simulink model "Plant"  (R2018b)
settings: configuration reference "plant_config" (kept outside this file)
values from neighbouring files (symbols this model uses):
  ada =     [acdata.mat]    (also in aero_data.mat)
  ade =     [acdata.mat]    (also in aero_data.mat)
  adr =     [acdata.mat]    (also in aero_data.mat)
  adyn =     [acdata.mat]    (also in aero_data.mat)
  alat =     [acdata.mat]    (also in aero_data.mat)
  alon =     [acdata.mat]    (also in aero_data.mat)
  geo =     [acdata.mat]    (also in aero_data.mat)
  mc =     [acdata.mat]    (also in aero_data.mat)
  PLANT_EXPORT = Simulink.Parameter(PLANT_EXPORT_VALUE)    [plant_model_init.m]
  PLANT_PARAM = Simulink.Parameter(PLANT_PARAM_VALUE)    [plant_model_init.m]
undefined symbols (not defined in the file or in its folder): acc_x, acc_x_O, acc_y, acc_y_O, acc_z, acc_z_O, alt, alt_0, day, diff_pressure, DiscIntNeverNeededParam, fixType, flags, gSpeed, gyr_x, gyr_y, gyr_z, h_R, hAcc, heading, headingAcc, height, hMSL, hour, iTOW, lat, lon, M_BO, M_OB, mag_x, mag_y, mag_z, month, nano, numSV, pDOP, phi, PLANT_CONST, plant_model, pressure, prop_vel, psi, quat, reserved1, reserved2, rot_x_B, rot_y_B, rot_z_B, sAcc, sec, Sensor_Model, tAcc, temperature, temprature, theta, timestamp, Va, vAcc, valid, vel_x_O ... (+8)
libraries: FMT_Model_Lib x23, simulink x14, dspsrcs4 x6, aerolibatmos2 x1
(part 1 of 3)
settings Model: Creator=jc  LastModifiedBy=zouji
settings ConfigSetRef: SourceLocation=Base Workspace

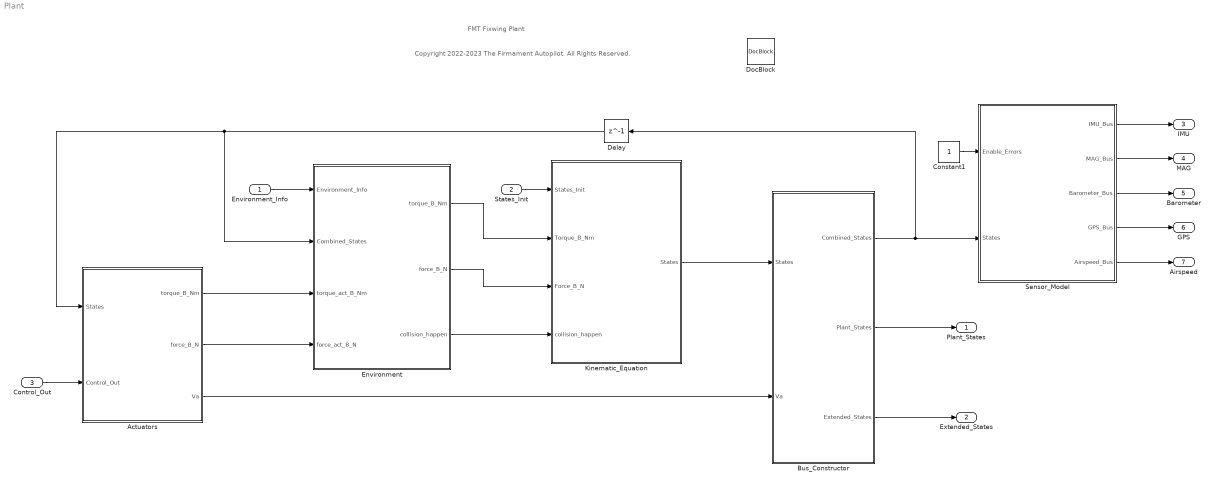
== system Plant ==
  note: FMT Fixwing Plant
  note: Copyright 2022-2023 The Firmament Autopilot. All Rights Reserved.
  Environment_Info : Inport  OutDataTypeStr=Bus: Environment_Info_Bus
  States_Init : Inport  Port=2  OutDataTypeStr=Bus: States_Init_Bus  Interpolate=off
  Control_Out : Inport  Port=3  OutDataTypeStr=Bus: Control_Out_Bus
  Actuators : Subsystem  TreatAsAtomicUnit=on
  Bus_Constructor : Subsystem  TreatAsAtomicUnit=on  mask{lat_0=PLANT_PARAM.LAT_0, lon_0=PLANT_PARAM.LON_0, hgt_0=PLANT_PARAM.ALT_0}
      mask prompts: lat_0 "init latitude (rad)"; lon_0 "init lontitude (rad)"; hgt_0 "init height (m)"
  Constant1 : Constant  OutDataTypeStr=Inherit: Inherit via back propagation
  Delay : Delay  DelayLength=1
  DocBlock : simulink/Model-Wide Utilities/DocBlock  DocumentType=Text
      content=|
      | This model is referenced from https://www.researchgate.net/publication/340630428_Guidance_and_control_for_a_fixed-wing_UAV
      | Aerodynamic data and models are contributed by pengyuan.shao@hotmail.com
  Environment : Subsystem  TreatAsAtomicUnit=on
  Kinematic_Equation : Subsystem  TreatAsAtomicUnit=on
  Sensor_Model : Subsystem  TreatAsAtomicUnit=on
  Plant_States : Outport  OutDataTypeStr=Bus: Plant_States_Bus
  Extended_States : Outport  Port=2  OutDataTypeStr=Bus: Extended_States_Bus
  IMU : Outport  Port=3  OutDataTypeStr=Bus: IMU_Bus
  MAG : Outport  Port=4  OutDataTypeStr=Bus: MAG_Bus
  Barometer : Outport  Port=5  OutDataTypeStr=Bus: Barometer_Bus
  GPS : Outport  Port=6  OutDataTypeStr=Bus: GPS_uBlox_Bus
  Airspeed : Outport  Port=7  OutDataTypeStr=Bus: AirSpeed_Bus
  wires:
  Environment/1(torque_B_Nm) -> Kinematic_Equation/2(Torque_B_Nm)
  Kinematic_Equation/1(States) -> Bus_Constructor/1(States)
  Actuators/2(force_B_N) -> Environment/4(force_act_B_N)
  Control_Out/1 -> Actuators/2(Control_Out)
  Actuators/1(torque_B_Nm) -> Environment/3(torque_act_B_Nm)
  Delay/1 -> Environment/2(Combined_States), Actuators/1(States)
  Environment/3(collision_happen) -> Kinematic_Equation/4(collision_happen)
  Environment/2(force_B_N) -> Kinematic_Equation/3(Force_B_N)
  Bus_Constructor/2(Plant_States) -> Plant_States/1
  Bus_Constructor/3(Extended_States) -> Extended_States/1
  Bus_Constructor/1(Combined_States) -> Delay/1, Sensor_Model/2(States)
  Sensor_Model/4(GPS_Bus) -> GPS/1
  Constant1/1 -> Sensor_Model/1(Enable_Errors)
  Sensor_Model/3(Barometer_Bus) -> Barometer/1
  Sensor_Model/2(MAG_Bus) -> MAG/1
  Sensor_Model/1(IMU_Bus) -> IMU/1
  Actuators/3(Va) -> Bus_Constructor/2(Va)
  Sensor_Model/5(Airspeed_Bus) -> Airspeed/1
  Environment_Info/1 -> Environment/1(Environment_Info)
  States_Init/1 -> Kinematic_Equation/1(States_Init)

== system Plant/Actuators ==
  States : Inport
  Control_Out : Inport  Port=2
  Aerodynamics Forces and Moments : Subsystem
  Propulsion Forces and Moments : Subsystem
  Reshape : Reshape  OutputDimensionality=Column vector (2-D)
  Reshape1 : Reshape  OutputDimensionality=Column vector (2-D)
  Sum : Sum  Inputs=|++
  Sum1 : Sum  Inputs=|++
  Wind_Triangle : Subsystem
  selector : Subsystem
  torque_B_Nm : Outport
  force_B_N : Outport  Port=2
  Va : Outport  Port=3
  wires:
  Control_Out/1 -> Aerodynamics Forces and Moments/5(Control_Out), Propulsion Forces and Moments/1(Control_Out)
  States/1 -> selector/1(States), Wind_Triangle/1(States)
  Wind_Triangle/1(Va) -> Aerodynamics Forces and Moments/1(Va_B), Va/1
  Wind_Triangle/2(alpha) -> Aerodynamics Forces and Moments/2(alpha)
  Wind_Triangle/3(beta) -> Aerodynamics Forces and Moments/3(beta)
  Aerodynamics Forces and Moments/2(Moment_B) -> Sum/1
  Propulsion Forces and Moments/2(Moment_B) -> Sum/2
  Sum/1 -> Reshape1/1
  Sum1/1 -> Reshape/1
  Aerodynamics Forces and Moments/1(Force_B) -> Sum1/1
  Propulsion Forces and Moments/1(Force_B) -> Sum1/2  "motor_force"
  Reshape/1 -> force_B_N/1
  Reshape1/1 -> torque_B_Nm/1
  selector/1(pqr) -> Aerodynamics Forces and Moments/4(pqr)

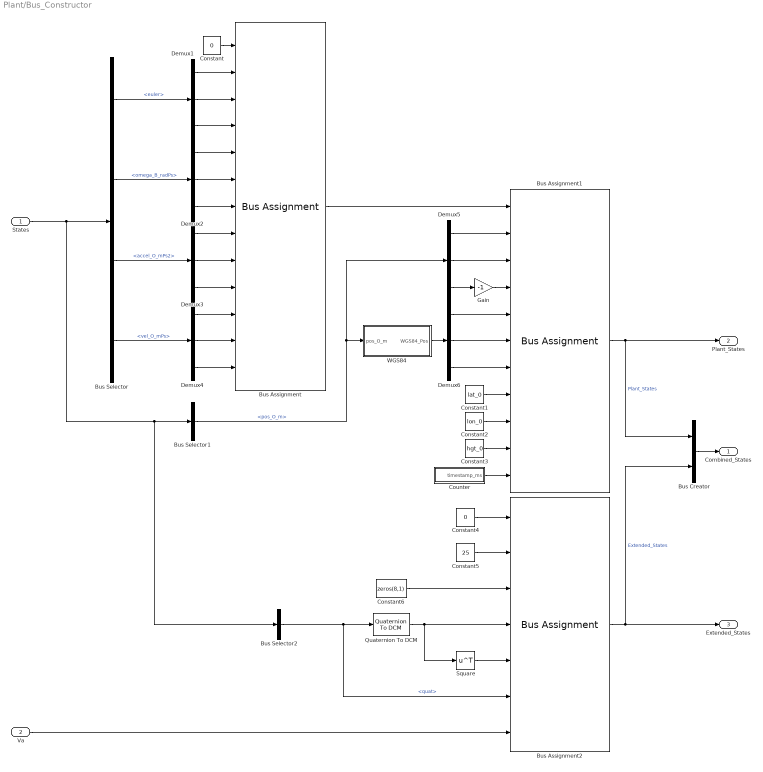
== system Plant/Bus_Constructor ==
  States : Inport
  Va : Inport  Port=2
  Bus Assignment : BusAssignment  AssignedSignals=phi,theta,psi,rot_x_B,rot_y_B,rot_z_B,acc_x_O,acc_y_O,acc_z_O,vel_x_O,vel_y_O,vel_z_O
  Bus Assignment1 : BusAssignment  AssignedSignals=x_R,y_R,h_R,lat,lon,alt,lat_0,lon_0,alt_0,timestamp
  Bus Assignment2 : BusAssignment  AssignedSignals=temprature,prop_vel,M_BO,M_OB,quat,Va
  Bus Creator : BusCreator  Inputs=2
  Bus Selector : BusSelector  OutputSignals=euler,omega_B_radPs,accel_O_mPs2,vel_O_mPs
  Bus Selector1 : BusSelector  OutputSignals=pos_O_m
  Bus Selector2 : BusSelector  OutputSignals=quat
  Constant : Constant  Value=0  OutDataTypeStr=Bus: Plant_States_Bus
  Constant1 : Constant  Value=lat_0
  Constant2 : Constant  Value=lon_0
  Constant3 : Constant  Value=hgt_0
  Constant4 : Constant  Value=0  OutDataTypeStr=Bus: Extended_States_Bus
  Constant5 : Constant  Value=25  OutDataTypeStr=Inherit: Inherit via back propagation
  Constant6 : Constant  Value=zeros(8,1)  OutDataTypeStr=single
  Counter : Subsystem
  Demux{1..6} (6 alike) : Demux  Outputs=3
  Gain : Gain  Gain=-1  OutDataTypeStr=Inherit: Same as input
  Quaternion To DCM : FMT_Model_Lib/Quaternion/Quaternion To DCM
      settings: SourceProductName=FMT Toolbox
  Square : Math  Operator=transpose  SaturateOnIntegerOverflow=on
  WGS84 : Subsystem
  Combined_States : Outport
  Plant_States : Outport  Port=2
  Extended_States : Outport  Port=3
  wires:
  Constant/1 -> Bus Assignment/1
  States/1 -> Bus Selector2/1, Bus Selector1/1, Bus Selector/1
  Bus Selector/1 -> Demux1/1  "<euler>"
  Bus Selector/2 -> Demux2/1  "<omega_B_radPs>"
  Bus Selector/3 -> Demux3/1  "<accel_O_mPs2>"
  Bus Selector/4 -> Demux4/1  "<vel_O_mPs>"
  Bus Assignment/1 -> Bus Assignment1/1
  Bus Selector1/1 -> Demux5/1, WGS84/1(pos_O_m)  "<pos_O_m>"
  Bus Assignment1/1 -> Plant_States/1, Bus Creator/1  "Plant_States"
  Demux1/2 -> Bus Assignment/3
  Demux5/3 -> Gain/1
  WGS84/1(WGS84_Pos) -> Demux6/1
  Demux1/1 -> Bus Assignment/2
  Demux1/3 -> Bus Assignment/4
  Demux2/1 -> Bus Assignment/5
  Demux2/2 -> Bus Assignment/6
  Demux2/3 -> Bus Assignment/7
  Demux3/1 -> Bus Assignment/8
  Demux3/2 -> Bus Assignment/9
  Demux3/3 -> Bus Assignment/10
  Demux4/1 -> Bus Assignment/11
  Demux4/2 -> Bus Assignment/12
  Demux4/3 -> Bus Assignment/13
  Demux5/2 -> Bus Assignment1/3
  Gain/1 -> Bus Assignment1/4
  Demux5/1 -> Bus Assignment1/2
  Demux6/1 -> Bus Assignment1/5
  Demux6/2 -> Bus Assignment1/6
  Demux6/3 -> Bus Assignment1/7
  Constant2/1 -> Bus Assignment1/9
  Constant1/1 -> Bus Assignment1/8
  Constant3/1 -> Bus Assignment1/10
  Constant4/1 -> Bus Assignment2/1
  Constant5/1 -> Bus Assignment2/2
  Constant6/1 -> Bus Assignment2/3
  Bus Selector2/1 -> Quaternion To DCM/1, Bus Assignment2/6  "<quat>"
  Bus Assignment2/1 -> Bus Creator/2, Extended_States/1  "Extended_States"
  Bus Creator/1 -> Combined_States/1
  Counter/1(timestamp_ms) -> Bus Assignment1/11
  Square/1 -> Bus Assignment2/5
  Quaternion To DCM/1 -> Square/1, Bus Assignment2/4
  Va/1 -> Bus Assignment2/7

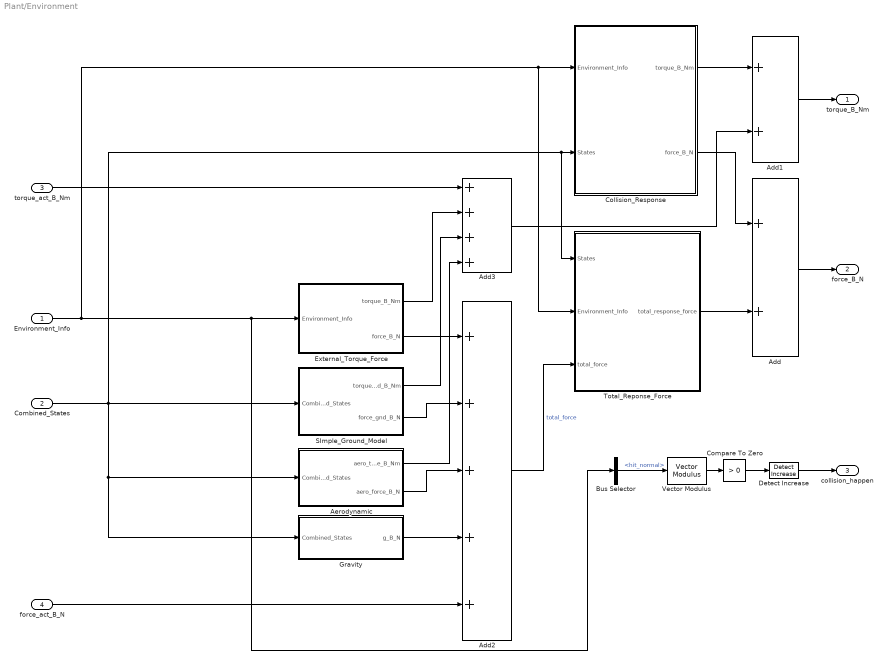
== system Plant/Environment ==
  Environment_Info : Inport
  Combined_States : Inport  Port=2
  torque_act_B_Nm : Inport  Port=3
  force_act_B_N : Inport  Port=4
  Add : Sum
  Add1 : Sum
  Add2 : Sum  Inputs=+++++
  Add3 : Sum  Inputs=++++
  Aerodynamic : Subsystem
  Bus Selector : BusSelector  OutputSignals=hit_normal
  Collision_Response : Subsystem  mask{e=0.5, u=1, Ixx=plant_model.Jxx, Iyy=plant_model.Jyy, Izz=plant_model.Jzz, m=plant_model.mass, dt=PLANT_CONST.dt}
      mask prompts: e "restitution coefficient [0 1]"; u "friction coefficient [0 1]"; m "mass (kg)"; dt "period (s)"
  Compare To Zero : simulink/Logic and Bit Operations/Compare To Zero  relop=>  OutDataTypeStr=boolean
  Detect Increase : simulink/Logic and Bit Operations/Detect Increase  vinit=0.0  OutDataTypeStr=boolean
  External_Torque_Force : Subsystem
  Gravity : Subsystem
  SImple_Ground_Model : Subsystem
  Total_Reponse_Force : Subsystem
  Vector Modulus : FMT_Model_Lib/Math/Vector Modulus
      settings: SourceProductName=FMT Toolbox
  torque_B_Nm : Outport
  force_B_N : Outport  Port=2
  collision_happen : Outport  Port=3
  wires:
  Add/1 -> force_B_N/1
  torque_act_B_Nm/1 -> Add3/1
  Add1/1 -> torque_B_Nm/1
  Combined_States/1 -> SImple_Ground_Model/1(Combined_States), Total_Reponse_Force/1(States), Collision_Response/2(States), Gravity/1(Combined_States), Aerodynamic/1(Combined_States)
  External_Torque_Force/2(force_B_N) -> Add2/1
  SImple_Ground_Model/2(force_gnd_B_N) -> Add2/2
  Gravity/1(g_B_N) -> Add2/4
  Aerodynamic/2(aero_force_B_N) -> Add2/3
  force_act_B_N/1 -> Add2/5
  SImple_Ground_Model/1(torque_gnd_B_Nm) -> Add3/3
  External_Torque_Force/1(torque_B_Nm) -> Add3/2
  Total_Reponse_Force/1(total_response_force) -> Add/2
  Add2/1 -> Total_Reponse_Force/3(total_force)  "total_force"
  Collision_Response/2(force_B_N) -> Add/1
  Add3/1 -> Add1/2
  Collision_Response/1(torque_B_Nm) -> Add1/1
  Aerodynamic/1(aero_torque_B_Nm) -> Add3/4
  Compare To Zero/1 -> Detect Increase/1
  Environment_Info/1 -> Bus Selector/1, External_Torque_Force/1(Environment_Info), Total_Reponse_Force/2(Environment_Info), Collision_Response/1(Environment_Info)
  Vector Modulus/1 -> Compare To Zero/1
  Bus Selector/1 -> Vector Modulus/1  "<hit_normal>"
  Detect Increase/1 -> collision_happen/1

== system Plant/Kinematic_Equation ==
  States_Init : Inport
  Torque_B_Nm : Inport  Port=2
  Force_B_N : Inport  Port=3
  collision_happen : Inport  Port=4
  Attitude_Dynamic : Subsystem  mask{Ixx=plant_model.Jxx, Iyy=plant_model.Jyy, Izz=plant_model.Jzz}
  Bus Creator : BusCreator  Inputs=7
  Constant : Constant  Value=0  OutDataTypeStr=Inherit: Inherit via back propagation
  Position_Dynamic : Subsystem  mask{mass=plant_model.mass}
  States : Outport
  wires:
  Attitude_Dynamic/2(omega_B_radPs) -> Position_Dynamic/2(omega_B_radPs), Bus Creator/2  "omega_B_radPs"
  Attitude_Dynamic/3(quat) -> Position_Dynamic/3(quat), Bus Creator/3  "quat"
  collision_happen/1 -> Position_Dynamic/4(vel_reset)
  Bus Creator/1 -> States/1  "states"
  Attitude_Dynamic/1(dot_omega_B_radPs2) -> Bus Creator/1  "dot_omega_B_radPs2"
  Attitude_Dynamic/4(euler) -> Bus Creator/4  "euler"
  Position_Dynamic/1(accel_O_mPs2) -> Bus Creator/5  "accel_O_mPs2"
  Position_Dynamic/2(vel_O_mPs) -> Bus Creator/6  "vel_O_mPs"
  Position_Dynamic/3(pos_O_m) -> Bus Creator/7  "pos_O_m"
  Force_B_N/1 -> Position_Dynamic/1(force_B_N)
  Torque_B_Nm/1 -> Attitude_Dynamic/1(torque_B_Nm)
  Constant/1 -> Attitude_Dynamic/2(rate_reset)
  States_Init/1 -> Position_Dynamic/5(States_Init), Attitude_Dynamic/3(States_Init)

== system Plant/Sensor_Model ==
  Enable_Errors : Inport  OutDataTypeStr=uint8
  States : Inport  Port=2
  Counter : Subsystem
  Sensor_Airspeed : Subsystem  TreatAsAtomicUnit=on
  Sensor_Barometer : Subsystem  TreatAsAtomicUnit=on
  Sensor_GPS : Subsystem  TreatAsAtomicUnit=on
  Sensor_IMU : Subsystem  TreatAsAtomicUnit=on
  Sensor_MAG : Subsystem  TreatAsAtomicUnit=on
  IMU_Bus : Outport
  MAG_Bus : Outport  Port=2
  Barometer_Bus : Outport  Port=3
  GPS_Bus : Outport  Port=4
  Airspeed_Bus : Outport  Port=5
  wires:
  Counter/1(timestamp_ms) -> Sensor_Airspeed/3(timestamp_ms), Sensor_Barometer/3(timestamp_ms), Sensor_MAG/3(timestamp_ms), Sensor_IMU/3(timestamp_ms), Sensor_GPS/3(timestamp_ms)
  States/1 -> Sensor_Airspeed/1(States), Sensor_GPS/1(States), Sensor_Barometer/1(States), Sensor_MAG/1(States), Sensor_IMU/1(States)
  Sensor_Barometer/1(Barometer_Bus) -> Barometer_Bus/1
  Sensor_MAG/1(MAG_Bus) -> MAG_Bus/1
  Sensor_IMU/1(IMU_Bus) -> IMU_Bus/1
  Enable_Errors/1 -> Sensor_IMU/2(Enable_Errors), Sensor_Airspeed/2(Enable_Errors), Sensor_GPS/2(Enable_Errors), Sensor_Barometer/2(Enable_Errors), Sensor_MAG/2(Enable_Errors)
  Sensor_GPS/1(GPS_Bus) -> GPS_Bus/1
  Sensor_Airspeed/1(Airspeed_Bus) -> Airspeed_Bus/1

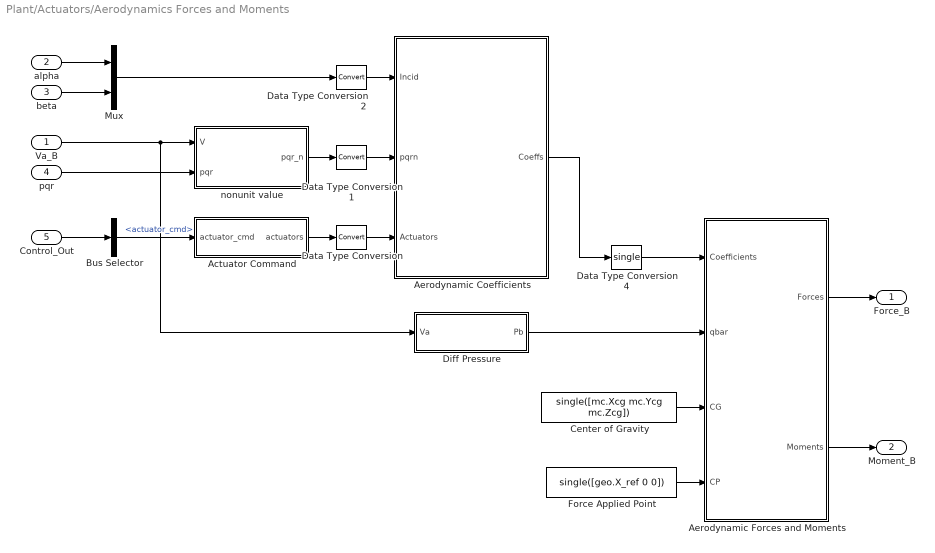
== system Plant/Actuators/Aerodynamics Forces and Moments ==
  Va_B : Inport
  alpha : Inport  Port=2
  beta : Inport  Port=3
  pqr : Inport  Port=4
  Control_Out : Inport  Port=5
  Actuator Command : Subsystem
  Aerodynamic Coefficients : Subsystem
  Aerodynamic Forces and Moments : Subsystem  mask(Aerodynamic Forces and Moments){S=geo.Sw, b=geo.b, cbar=geo.MAC}
      mask prompts: S "Reference area:"; b "Reference span:"; cbar "Reference length:"
      mask help: Compute the aerodynamic forces and moments applied at the center of gravity using the aerodynamic coefficients, dynamic pressure, center of gravity and center of pressure.
      mask Help: web(asbhelp);
      mask Display:
      | port_label('input',1,'Coefficients','texmode','on');
      | port_label('input',2,'q_{bar}','texmode','on');
      | port_label('input',3,'CG','texmode','on');
      | port_label('input',4,'CP','texmode','on');
      | port_label('output',1,'F_{aero}','texmode','on');
      | port_label('output',2,'M_{aero}','texmode','on');
  Bus Selector : BusSelector  OutputSignals=actuator_cmd
  Center of Gravity : Constant  Value=single([mc.Xcg mc.Ycg mc.Zcg])
  Data Type Conversion : DataTypeConversion
  Data Type Conversion1 : DataTypeConversion
  Data Type Conversion2 : DataTypeConversion
  Data Type Conversion4 : DataTypeConversion  OutDataTypeStr=single
  Diff Pressure : Subsystem
  Force Applied Point : Constant  Value=single([geo.X_ref 0 0])
  Mux : Mux  Inputs=2
  nonunit value : Subsystem
  Force_B : Outport
  Moment_B : Outport  Port=2
  wires:
  Control_Out/1 -> Bus Selector/1
  nonunit value/1(pqr_n) -> Data Type Conversion1/1
  Mux/1 -> Data Type Conversion2/1
  alpha/1 -> Mux/1
  beta/1 -> Mux/2
  Va_B/1 -> Diff Pressure/1(Va), nonunit value/1(V)
  pqr/1 -> nonunit value/2(pqr)
  Bus Selector/1 -> Actuator Command/1(actuator_cmd)  "<actuator_cmd>"
  Actuator Command/1(actuators) -> Data Type Conversion/1
  Data Type Conversion/1 -> Aerodynamic Coefficients/3(Actuators)
  Data Type Conversion1/1 -> Aerodynamic Coefficients/2(pqrn)
  Data Type Conversion2/1 -> Aerodynamic Coefficients/1(Incid)
  Aerodynamic Coefficients/1(Coeffs) -> Data Type Conversion4/1
  Data Type Conversion4/1 -> Aerodynamic Forces and Moments/1(Coefficients)
  Aerodynamic Forces and Moments/2(Moments) -> Moment_B/1
  Aerodynamic Forces and Moments/1(Forces) -> Force_B/1
  Center of Gravity/1 -> Aerodynamic Forces and Moments/3(CG)
  Force Applied Point/1 -> Aerodynamic Forces and Moments/4(CP)
  Diff Pressure/1(Pb) -> Aerodynamic Forces and Moments/2(qbar)

== system Plant/Actuators/Propulsion Forces and Moments ==
  Control_Out : Inport
  Constant : Constant  Value=[0 0 0]  OutDataTypeStr=single
  ESCs : Subsystem  mask{T=plant_model.motorT, k=plant_model.motorCr, p=plant_model.motorWb}
  Force : Subsystem
  Force_B : Outport
  Moment_B : Outport  Port=2
  wires:
  ESCs/1(rotor_speed_radPs) -> Force/1(rotor_speed_radPs)
  Control_Out/1 -> ESCs/1(Control_Out)
  Constant/1 -> Moment_B/1
  Force/1(force_B_N) -> Force_B/1

== system Plant/Actuators/Wind_Triangle ==
  States : Inport
  Attack_Angle : Subsystem
  Bus Selector : BusSelector  OutputSignals=Plant_States.vel_x_O,Plant_States.vel_y_O,Plant_States.vel_z_O
  Bus Selector1 : BusSelector  OutputSignals=Extended_States.M_BO
  Multiply : Product  Multiplication=Matrix(*)
  Mux : Mux  Inputs=3
  Selector : Selector  InputPortWidth=3  IndexOptions=Index vector (dialog)  Indices=1  OutputSizes=1
  Slide_Angle : Subsystem
  Sum : Sum  Inputs=|+-
  Wind_Velocity_O : Constant  Value=[0;0;0]  VectorParams1D=off  OutDataTypeStr=single
  Va : Outport
  alpha : Outport  Port=2
  beta : Outport  Port=3
  wires:
  States/1 -> Bus Selector1/1, Bus Selector/1
  Bus Selector/1 -> Mux/1  "<vel_x_O>"
  Bus Selector/2 -> Mux/2  "<vel_y_O>"
  Bus Selector/3 -> Mux/3  "<vel_z_O>"
  Bus Selector1/1 -> Multiply/1  "<M_BO>"
  Multiply/1 -> Selector/1, Slide_Angle/1(Va_B), Attack_Angle/1(Va_B)  "Va_B"
  Attack_Angle/1(alpha_rad) -> alpha/1  "alpha_rad"
  Slide_Angle/1(beta_rad) -> beta/1  "beta_rad"
  Selector/1 -> Va/1
  Mux/1 -> Sum/1
  Sum/1 -> Multiply/2
  Wind_Velocity_O/1 -> Sum/2

== system Plant/Actuators/selector ==
  States : Inport
  Bus Selector : BusSelector  OutputSignals=Plant_States.rot_x_B,Plant_States.rot_y_B,Plant_States.rot_z_B
  Mux : Mux  Inputs=3
  pqr : Outport
  wires:
  Bus Selector/1 -> Mux/1  "<rot_x_B>"
  Bus Selector/3 -> Mux/3  "<rot_z_B>"
  Bus Selector/2 -> Mux/2  "<rot_y_B>"
  Mux/1 -> pqr/1
  States/1 -> Bus Selector/1

== system Plant/Bus_Constructor/Counter ==
  Data Type Conversion2 : DataTypeConversion  OutDataTypeStr=uint32
  Delay : Delay  DelayLength=1  InitialCondition=0
  Sum : Sum  Inputs=|++
  dt : Constant  Value=PLANT_EXPORT.period  OutDataTypeStr=uint32
  timestamp_ms : Outport
  wires:
  dt/1 -> Sum/1
  Sum/1 -> Delay/1
  Delay/1 -> Data Type Conversion2/1
  Data Type Conversion2/1 -> timestamp_ms/1, Sum/2

== system Plant/Bus_Constructor/WGS84 ==
  pos_O_m : Inport
  Add : Sum
  Constant1 : Constant  Value=lat_0
  Constant2 : Constant  Value=lon_0
  Constant3 : Constant  Value=hgt_0
  Data Type Conversion : DataTypeConversion  OutDataTypeStr=double
  Delay : Delay  DelayLength=1
  Delay1 : Delay  DelayLength=1  InitialConditionSource=Input port  InitialCondition=[lat_0;lon_0;hgt_0]
      settings: InputPortMap=u0,p4
  Demux : Demux  Outputs=3
  Divide : Product  Inputs=/*
  Mux : Mux  Inputs=3
  Mux1 : Mux  Inputs=3
  Subtract : Sum  Inputs=+-
  Terminator : Terminator
  WGS84_Derivative : Subsystem
  Zero_Value_Exclusion : Subsystem
  WGS84_Pos : Outport
  wires:
  pos_O_m/1 -> Data Type Conversion/1
  Delay/1 -> Subtract/2
  WGS84_Derivative/1(dx_dlat) -> Mux/1
  Mux/1 -> Zero_Value_Exclusion/1(u)
  Zero_Value_Exclusion/1(y) -> Divide/1
  WGS84_Derivative/3(dz_dh) -> Mux/3
  WGS84_Derivative/2(dy_dlon) -> Mux/2
  Subtract/1 -> Divide/2
  Divide/1 -> Add/1
  Delay1/1 -> Demux/1, Add/2
  Demux/1 -> WGS84_Derivative/1(lat_0)
  Demux/3 -> WGS84_Derivative/2(h_0)
  Demux/2 -> Terminator/1
  Data Type Conversion/1 -> Delay/1, Subtract/1
  Constant1/1 -> Mux1/1
  Mux1/1 -> Delay1/2
  Add/1 -> Delay1/1, WGS84_Pos/1
  Constant2/1 -> Mux1/2
  Constant3/1 -> Mux1/3

== system Plant/Environment/Aerodynamic ==
  Combined_States : Inport
  Air_Drag : Subsystem
  aero_torque_B_Nm : Outport
  aero_force_B_N : Outport  Port=2
  wires:
  Combined_States/1 -> Air_Drag/1(Combined_States)
  Air_Drag/2(airdrag_force_B) -> aero_force_B_N/1  "aero_force_B_N"
  Air_Drag/1(airdrag_torque_B) -> aero_torque_B_Nm/1  "aero_torque_B_N"

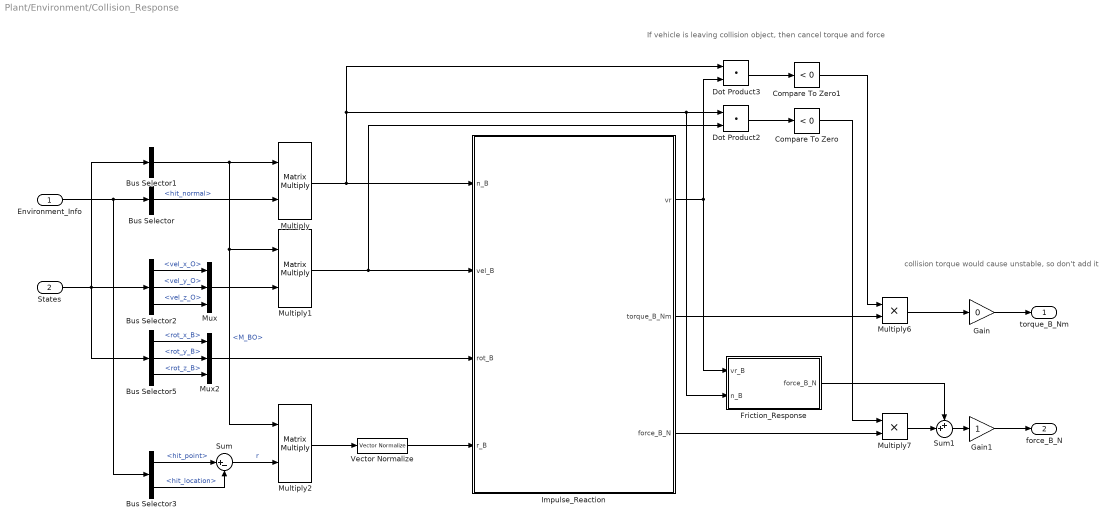
== system Plant/Environment/Collision_Response ==
  note: collision torque would cause unstable, so don't add it
  note: If vehicle is leaving collision object, then cancel torque and force
  Environment_Info : Inport
  States : Inport  Port=2
  Bus Selector : BusSelector  OutputSignals=hit_normal
  Bus Selector1 : BusSelector  OutputSignals=Extended_States.M_BO
  Bus Selector2 : BusSelector  OutputSignals=Plant_States.vel_x_O,Plant_States.vel_y_O,Plant_States.vel_z_O
  Bus Selector3 : BusSelector  OutputSignals=hit_point,hit_location
  Bus Selector5 : BusSelector  OutputSignals=Plant_States.rot_x_B,Plant_States.rot_y_B,Plant_States.rot_z_B
  Compare To Zero : simulink/Logic and Bit Operations/Compare To Zero  relop=<  OutDataTypeStr=boolean
  Compare To Zero1 : simulink/Logic and Bit Operations/Compare To Zero  relop=<  OutDataTypeStr=boolean
  Dot Product2 : DotProduct  InputSameDT=on  OutDataTypeStr=Inherit: Inherit via internal rule
  Dot Product3 : DotProduct  InputSameDT=on  OutDataTypeStr=Inherit: Inherit via internal rule
  Friction_Response : Subsystem
  Gain : Gain  Gain=0
  Gain1 : Gain
  Impulse_Reaction : Subsystem
  Multiply : Product  Multiplication=Matrix(*)
  Multiply1 : Product  Multiplication=Matrix(*)
  Multiply2 : Product  Multiplication=Matrix(*)
  Multiply6 : Product
  Multiply7 : Product
  Mux : Mux  Inputs=3
  Mux2 : Mux  Inputs=3
  Sum : Sum  Inputs=|+-
  Sum1 : Sum  Inputs=++|
  Vector Normalize : FMT_Model_Lib/Math/Vector Normalize
      settings: SourceProductName=FMT Toolbox
  torque_B_Nm : Outport
  force_B_N : Outport  Port=2
  wires:
  Environment_Info/1 -> Bus Selector3/1, Bus Selector/1
  Bus Selector/1 -> Multiply/2  "<hit_normal>"
  States/1 -> Bus Selector1/1, Bus Selector5/1, Bus Selector2/1
  Bus Selector1/1 -> Multiply/1, Multiply2/1, Multiply1/1  "<M_BO>"
  Bus Selector2/1 -> Mux/1  "<vel_x_O>"
  Bus Selector2/2 -> Mux/2  "<vel_y_O>"
  Bus Selector2/3 -> Mux/3  "<vel_z_O>"
  Mux/1 -> Multiply1/2
  Multiply1/1 -> Dot Product2/2, Impulse_Reaction/2(vel_B)
  Bus Selector3/1 -> Sum/1  "<hit_point>"
  Multiply2/1 -> Vector Normalize/1
  Bus Selector5/2 -> Mux2/2  "<rot_y_B>"
  Bus Selector5/3 -> Mux2/3  "<rot_z_B>"
  Bus Selector5/1 -> Mux2/1  "<rot_x_B>"
  Multiply/1 -> Dot Product2/1, Friction_Response/2(n_B), Dot Product3/1, Impulse_Reaction/1(n_B)
  Dot Product2/1 -> Compare To Zero/1
  Compare To Zero/1 -> Multiply7/1
  Multiply6/1 -> Gain/1
  Multiply7/1 -> Sum1/2
  Dot Product3/1 -> Compare To Zero1/1
  Compare To Zero1/1 -> Multiply6/1
  Bus Selector3/2 -> Sum/2  "<hit_location>"
  Sum/1 -> Multiply2/2  "r"
  Mux2/1 -> Impulse_Reaction/3(rot_B)
  Vector Normalize/1 -> Impulse_Reaction/4(r_B)
  Impulse_Reaction/1(vr) -> Dot Product3/2, Friction_Response/1(vr_B)
  Impulse_Reaction/2(torque_B_Nm) -> Multiply6/2
  Impulse_Reaction/3(force_B_N) -> Multiply7/2
  Friction_Response/1(force_B_N) -> Sum1/1
  Gain/1 -> torque_B_Nm/1
  Gain1/1 -> force_B_N/1
  Sum1/1 -> Gain1/1

== system Plant/Environment/External_Torque_Force ==
  Environment_Info : Inport
  Bus Selector : BusSelector  OutputSignals=torque,force
  torque_B_Nm : Outport
  force_B_N : Outport  Port=2
  wires:
  Environment_Info/1 -> Bus Selector/1
  Bus Selector/1 -> torque_B_Nm/1  "<torque>"
  Bus Selector/2 -> force_B_N/1  "<force>"

== system Plant/Environment/Gravity ==
  Combined_States : Inport
  Bus Selector4 : BusSelector  OutputSignals=Extended_States.M_BO
  Multiply3 : Product  Multiplication=Matrix(*)
  mg : Constant  Value=[0;0;9.81*plant_model.mass]  OutDataTypeStr=single
  g_B_N : Outport
  wires:
  Combined_States/1 -> Bus Selector4/1
  Bus Selector4/1 -> Multiply3/1  "<M_BO>"
  Multiply3/1 -> g_B_N/1
  mg/1 -> Multiply3/2

== system Plant/Environment/SImple_Ground_Model ==
  Combined_States : Inport
  Bus Selector : BusSelector  OutputSignals=Plant_States.h_R
  Compare To Zero : simulink/Logic and Bit Operations/Compare To Zero  relop=<  OutDataTypeStr=boolean
  Constant : Constant  Value=[0;0;0]  VectorParams1D=off  OutDataTypeStr=single
  Constant1 : Constant  Value=[0;0;0]  VectorParams1D=off  OutDataTypeStr=single
  Ground_Force : Subsystem
  Ground_Torque : Subsystem
  Switch1 : Switch  Criteria=u2 > Threshold
  Switch2 : Switch  Criteria=u2 > Threshold
  torque_gnd_B_Nm : Outport
  force_gnd_B_N : Outport  Port=2
  wires:
  Compare To Zero/1 -> Switch1/2, Switch2/2
  Constant/1 -> Switch2/3
  Switch2/1 -> force_gnd_B_N/1
  Combined_States/1 -> Ground_Force/1(Combined_States), Bus Selector/1, Ground_Torque/1(States)
  Bus Selector/1 -> Compare To Zero/1  "<h_R>"
  Ground_Force/1(force_gnd_B_N) -> Switch2/1
  Ground_Torque/1(torque_gnd_B_Nm) -> Switch1/1
  Constant1/1 -> Switch1/3
  Switch1/1 -> torque_gnd_B_Nm/1

== system Plant/Environment/Total_Reponse_Force ==
  States : Inport
  Environment_Info : Inport  Port=2
  total_force : Inport  Port=3
  Bus Selector : BusSelector  OutputSignals=hit_normal
  Bus Selector1 : BusSelector  OutputSignals=Extended_States.M_BO
  Compare To Zero : simulink/Logic and Bit Operations/Compare To Zero  relop=<  OutDataTypeStr=boolean
  Dot Product : DotProduct  InputSameDT=on  OutDataTypeStr=Inherit: Inherit via internal rule
  Multiply : Product  Multiplication=Matrix(*)
  Multiply1 : Product  Inputs=3
  Sum : Sum  Inputs=|+-
  total_response_force : Outport
  wires:
  total_force/1 -> Dot Product/1, Sum/1
  Bus Selector/1 -> Multiply/2  "<hit_normal>"
  Bus Selector1/1 -> Multiply/1  "<M_BO>"
  Multiply/1 -> Multiply1/3, Dot Product/2  "n_B"
  States/1 -> Bus Selector1/1
  Environment_Info/1 -> Bus Selector/1
  Multiply1/1 -> Sum/2
  Sum/1 -> total_response_force/1
  Compare To Zero/1 -> Multiply1/1
  Dot Product/1 -> Multiply1/2, Compare To Zero/1

== system Plant/Kinematic_Equation/Attitude_Dynamic ==
  torque_B_Nm : Inport
  rate_reset : Inport  Port=2
  States_Init : Inport  Port=3
  Bus Selector : BusSelector  OutputSignals=timestamp,euler
  Cross Product : FMT_Model_Lib/Math/Cross Product
      settings: SourceProductName=FMT Toolbox
  Detect Change : simulink/Logic and Bit Operations/Detect Change  vinit=0  OutDataTypeStr=boolean
  Discrete-Time Integrator : DiscreteIntegrator  ExternalReset=level  InitialCondition=[0;0;0]  SampleTime=-1  ICPrevOutput=DiscIntNeverNeededParam  ICPrevScaledInput=DiscIntNeverNeededParam
  Divide : Product  Inputs=/*  Multiplication=Matrix(*)  OutDataTypeStr=Inherit: Same as first input
  Euler To Quaternion : FMT_Model_Lib/Quaternion/Euler To Quaternion
      settings: SourceProductName=FMT Toolbox
  Inertia_Matrix : Constant  Value=[Ixx 0 0;0 Iyy 0;0 0 Izz]  OutDataTypeStr=single
  Logical Operator : Logic  Operator=OR  AllPortsSameDT=off  OutDataTypeStr=boolean
  Multiply : Product  Multiplication=Matrix(*)  OutDataTypeStr=Inherit: Same as first input
  Quaternion To Euler : FMT_Model_Lib/Quaternion/Quaternion To Euler
      settings: SourceProductName=FMT Toolbox
  Quaternuin_Update : Subsystem
  Sum : Sum  Inputs=|+-  OutDataTypeStr=Inherit: Same as first input
  dot_omega_B_radPs2 : Outport
  omega_B_radPs : Outport  Port=2
  quat : Outport  Port=3
  euler : Outport  Port=4
  wires:
  Quaternion To Euler/1 -> euler/1
  Quaternuin_Update/1(quat) -> Quaternion To Euler/1, quat/1
  rate_reset/1 -> Logical Operator/1
  Divide/1 -> dot_omega_B_radPs2/1, Discrete-Time Integrator/1  "dot_omega_B_radPs2"
  Sum/1 -> Divide/2
  Cross Product/1 -> Sum/2
  torque_B_Nm/1 -> Sum/1
  Multiply/1 -> Cross Product/2
  Inertia_Matrix/1 -> Multiply/1, Divide/1
  Discrete-Time Integrator/1 -> omega_B_radPs/1, Cross Product/1, Multiply/2, Quaternuin_Update/1(omega_B_radPs)  "omega_B_radPs"
  States_Init/1 -> Bus Selector/1
  Bus Selector/1 -> Detect Change/1  "<timestamp>"
  Logical Operator/1 -> Discrete-Time Integrator/2
  Detect Change/1 -> Quaternuin_Update/2(att_reset), Logical Operator/2
  Bus Selector/2 -> Euler To Quaternion/1  "<euler>"
  Euler To Quaternion/1 -> Quaternuin_Update/3(quat_0)

== system Plant/Kinematic_Equation/Position_Dynamic ==
  force_B_N : Inport
  omega_B_radPs : Inport  Port=2
  quat : Inport  Port=3
  vel_reset : Inport  Port=4
  States_Init : Inport  Port=5
  Bus Selector : BusSelector  OutputSignals=timestamp,pos
  Cross Product : FMT_Model_Lib/Math/Cross Product
      settings: SourceProductName=FMT Toolbox
  Detect Change : simulink/Logic and Bit Operations/Detect Change  vinit=0  OutDataTypeStr=boolean
  Discrete-Time Integrator : DiscreteIntegrator  ExternalReset=level  InitialCondition=[0;0;0]  SampleTime=-1  ICPrevOutput=DiscIntNeverNeededParam  ICPrevScaledInput=DiscIntNeverNeededParam
  Discrete-Time Integrator1 : DiscreteIntegrator  ExternalReset=level  InitialConditionSource=external  InitialCondition=[0;0;0]  SampleTime=-1  ICPrevOutput=DiscIntNeverNeededParam  ICPrevScaledInput=DiscIntNeverNeededParam
  Divide : Product  Inputs=*/
  Logical Operator : Logic  Operator=OR  AllPortsSameDT=off  OutDataTypeStr=boolean
  Quaternion Inv-Rotation : FMT_Model_Lib/Quaternion/Quaternion Inv-Rotation
      settings: SourceProductName=FMT Toolbox
  Quaternion Rotation : FMT_Model_Lib/Quaternion/Quaternion Rotation
      settings: SourceProductName=FMT Toolbox
  Sum : Sum  Inputs=|+-
  mass : Constant  Value=mass  OutDataTypeStr=single
  accel_O_mPs2 : Outport
  vel_O_mPs : Outport  Port=2
  pos_O_m : Outport  Port=3
  wires:
  force_B_N/1 -> Divide/1
  mass/1 -> Divide/2
  Discrete-Time Integrator/1 -> Quaternion Inv-Rotation/2, Discrete-Time Integrator1/1, vel_O_mPs/1  "vel_O_mPs"
  Divide/1 -> Sum/1
  Cross Product/1 -> Sum/2  "centripetal_accel"
  Sum/1 -> Quaternion Rotation/2
  quat/1 -> Quaternion Inv-Rotation/1, Quaternion Rotation/1
  Discrete-Time Integrator1/1 -> pos_O_m/1
  Quaternion Rotation/1 -> accel_O_mPs2/1, Discrete-Time Integrator/1  "accel_O_mPs2"
  Quaternion Inv-Rotation/1 -> Cross Product/2
  omega_B_radPs/1 -> Cross Product/1
  Logical Operator/1 -> Discrete-Time Integrator/2
  vel_reset/1 -> Logical Operator/1
  States_Init/1 -> Bus Selector/1
  Bus Selector/1 -> Detect Change/1  "<timestamp>"
  Detect Change/1 -> Discrete-Time Integrator1/2, Logical Operator/2
  Bus Selector/2 -> Discrete-Time Integrator1/3  "<pos>"

== system Plant/Sensor_Model/Counter ==
  Data Type Conversion2 : DataTypeConversion  OutDataTypeStr=uint32
  Memory1 : Memory
  Sum : Sum  Inputs=|++
  dt : Constant  Value=PLANT_EXPORT.period  OutDataTypeStr=uint32
  timestamp_ms : Outport
  wires:
  dt/1 -> Sum/1
  Sum/1 -> Memory1/1
  Memory1/1 -> Sum/2, Data Type Conversion2/1
  Data Type Conversion2/1 -> timestamp_ms/1

== system Plant/Sensor_Model/Sensor_Airspeed ==
  States : Inport
  Enable_Errors : Inport  Port=2
  timestamp_ms : Inport  Port=3
  Airspeed : Subsystem
  Bus_Constructor : Subsystem
  Airspeed_Bus : Outport
  wires:
  Bus_Constructor/1(Airspeed_Bus) -> Airspeed_Bus/1
  Enable_Errors/1 -> Airspeed/1(Enable_Errors)
  States/1 -> Airspeed/2(States)
  Airspeed/1(diff_pressure_Pa) -> Bus_Constructor/1(diff_pressure_Pa)
  timestamp_ms/1 -> Bus_Constructor/2(timestamp_ms)

== system Plant/Sensor_Model/Sensor_Barometer ==
  States : Inport
  Enable_Errors : Inport  Port=2
  timestamp_ms : Inport  Port=3
  Barometer : Subsystem
  Bus_Constructor : Subsystem
  Barometer_Bus : Outport
  wires:
  Bus_Constructor/1(Barometer_Bus) -> Barometer_Bus/1
  timestamp_ms/1 -> Bus_Constructor/3(timestamp_ms)
  Enable_Errors/1 -> Barometer/1(Enable_Errors)
  States/1 -> Barometer/2(States)
  Barometer/1(pressure_Pa) -> Bus_Constructor/1(pressure_Pa)
  Barometer/2(temprature_K) -> Bus_Constructor/2(temperature_K)

== system Plant/Sensor_Model/Sensor_GPS ==
  States : Inport
  Enable_Errors : Inport  Port=2
  timestamp_ms : Inport  Port=3
  Bus_Constructor : Subsystem
  GPS : Subsystem
  GPS_Bus : Outport
  wires:
  Bus_Constructor/1(GPS_Bus) -> GPS_Bus/1
  timestamp_ms/1 -> Bus_Constructor/2(timestamp_ms)
  Enable_Errors/1 -> GPS/1(Enable_Errors)
  States/1 -> GPS/2(States)
  GPS/1(GPS_Raw) -> Bus_Constructor/1(GPS_Raw)

== system Plant/Sensor_Model/Sensor_IMU ==
  States : Inport
  Enable_Errors : Inport  Port=2
  timestamp_ms : Inport  Port=3
  Accelerometer : Subsystem
  Bus_Constructor : Subsystem
  Gyroscope : Subsystem
  IMU_Bus : Outport
  wires:
  Gyroscope/1(Gyro_Raw) -> Bus_Constructor/1(Gyro_Raw)
  Bus_Constructor/1(IMU_Bus) -> IMU_Bus/1
  States/1 -> Gyroscope/1(States), Accelerometer/1(States)
  Enable_Errors/1 -> Gyroscope/2(Enable_Errors), Accelerometer/2(Enable_Errors)
  Accelerometer/1(Acc_Raw) -> Bus_Constructor/2(Acc_Raw)
  timestamp_ms/1 -> Bus_Constructor/3(timestamp_ms)

== system Plant/Sensor_Model/Sensor_MAG ==
  States : Inport
  Enable_Errors : Inport  Port=2
  timestamp_ms : Inport  Port=3
  Bus_Constructor : Subsystem
  Magnetometer : Subsystem
  MAG_Bus : Outport
  wires:
  Magnetometer/1(Mag_Raw) -> Bus_Constructor/1(Mag_Raw)
  Bus_Constructor/1(MAG_Bus) -> MAG_Bus/1
  States/1 -> Magnetometer/1(States)
  Enable_Errors/1 -> Magnetometer/2(Enable_Errors)
  timestamp_ms/1 -> Bus_Constructor/2(timestamp_ms)

== system Plant/Actuators/Aerodynamics Forces and Moments/Actuator Command ==
  actuator_cmd : Inport
  Mux1 : Mux  Inputs=3
  aileron_cmd : Subsystem
  elevator_cmd : Subsystem
  rudder_cmd : Subsystem
  actuators : Outport
  wires:
  elevator_cmd/1(elevator_cmd) -> Mux1/2
  rudder_cmd/1(rudder_cmd) -> Mux1/3
  Mux1/1 -> actuators/1
  aileron_cmd/1(aileron_cmd) -> Mux1/1
  actuator_cmd/1 -> rudder_cmd/1(actuator_cmd), aileron_cmd/1(actuator_cmd), elevator_cmd/1(actuator_cmd)

== system Plant/Actuators/Aerodynamics Forces and Moments/Aerodynamic Coefficients ==
  Incid : Inport
  pqrn : Inport  Port=2
  Actuators : Inport  Port=3
  Actuator increments : Subsystem
  Basic Coefficients : Subsystem
  Mux1 : Mux  Inputs=2
  Selector : Selector  InputPortWidth=6  IndexOptions=Index vector (dialog)  Indices=[1 2 3]  OutputSizes=1
  Selector1 : Selector  InputPortWidth=6  IndexOptions=Index vector (dialog)  Indices=[4 5 6]  OutputSizes=1
  Sum : Sum  Inputs=3  SaturateOnIntegerOverflow=on  InputSameDT=on  OutDataTypeStr=Inherit: Same as first input
  body axis forces : Subsystem
  body rate damping : Subsystem
  Coeffs : Outport  InitialOutput=0
  wires:
  Sum/1 -> Selector/1, Selector1/1
  Incid/1 -> body axis forces/1(Incid), Basic Coefficients/1(incid), body rate damping/1(Incid), Actuator increments/1(Incid)
  Selector1/1 -> Mux1/2  "C_LMN"
  Mux1/1 -> Coeffs/1
  Actuators/1 -> Actuator increments/2(ActData)
  pqrn/1 -> body rate damping/2(pqr_n)
  Basic Coefficients/1(Coeffs) -> Sum/1  "C_Basic"
  Actuator increments/1(Coeffs) -> Sum/3  "C_Inc"
  body rate damping/1(Coeffs) -> Sum/2  "C_damp"
  Selector/1 -> body axis forces/2(Cl_DLY)
  body axis forces/1(Cl_XYZ) -> Mux1/1  "C_XYZ"

== system Plant/Actuators/Aerodynamics Forces and Moments/Aerodynamic Forces and Moments ==
  Coefficients : Inport
  qbar : Inport  Port=2
  CG : Inport  Port=3
  CP : Inport  Port=4
  Demux1 : Demux  Outputs=[3,3]
  Moments about CG due to Forces : Subsystem
  Product : Product  SaturateOnIntegerOverflow=on  InputSameDT=on  OutDataTypeStr=Inherit: Same as first input
  Product3 : Product  SaturateOnIntegerOverflow=on  InputSameDT=on  OutDataTypeStr=Inherit: Same as first input
  Sum1 : Sum  Inputs=++|  SaturateOnIntegerOverflow=on  InputSameDT=on  OutDataTypeStr=Inherit: Same as first input
  reference area : Gain  Gain=S  SaturateOnIntegerOverflow=on  OutDataTypeStr=Inherit: Same as input  ParamDataTypeStr=Inherit: Same as input
  reference length : Gain  Gain=[b cbar b]  SaturateOnIntegerOverflow=on  OutDataTypeStr=Inherit: Same as input  ParamDataTypeStr=Inherit: Same as input
  Forces : Outport
  Moments : Outport  Port=2
  wires:
  CP/1 -> Moments about CG due to Forces/3(CP)
  CG/1 -> Moments about CG due to Forces/2(CG)
  Sum1/1 -> Moments/1
  Product3/1 -> Sum1/2
  Product/1 -> Moments about CG due to Forces/1(Forces), Forces/1
  reference area/1 -> Product/1, reference length/1
  qbar/1 -> reference area/1
  Demux1/2 -> Product3/1
  Demux1/1 -> Product/2
  Coefficients/1 -> Demux1/1
  reference length/1 -> Product3/2
  Moments about CG due to Forces/1(Moments) -> Sum1/1

== system Plant/Actuators/Aerodynamics Forces and Moments/Diff Pressure ==
  Va : Inport
  Gain : Gain  Gain=0.5*1.29
  Square : Math  Operator=square  SaturateOnIntegerOverflow=on
  Pb : Outport
  wires:
  Gain/1 -> Pb/1
  Square/1 -> Gain/1
  Va/1 -> Square/1

== system Plant/Actuators/Aerodynamics Forces and Moments/nonunit value ==
  V : Inport
  pqr : Inport  Port=2
  Demux2 : Demux  Outputs=3
  Gain : Gain  Gain=2  SaturateOnIntegerOverflow=on  OutDataTypeStr=Inherit: Same as input  ParamDataTypeStr=Inherit: Same as input
  Mux18 : Mux  Inputs=3
  Product1 : Product  Inputs=/**  SaturateOnIntegerOverflow=on  OutDataTypeStr=Inherit: Same as first input
  Product2 : Product  Inputs=/**  SaturateOnIntegerOverflow=on  OutDataTypeStr=Inherit: Same as first input
  Product4 : Product  Inputs=/**  SaturateOnIntegerOverflow=on  OutDataTypeStr=Inherit: Same as first input
  Saturation : Saturate  UpperLimit=inf  LowerLimit=0.1
  b : Constant  Value=geo.b  OutDataTypeStr=single
  c : Constant  Value=geo.MAC  OutDataTypeStr=single
  pqr_n : Outport
  wires:
  pqr/1 -> Demux2/1
  V/1 -> Gain/1
  Product4/1 -> Mux18/2
  Product2/1 -> Mux18/3
  Gain/1 -> Saturation/1
  b/1 -> Product1/2, Product2/2
  Demux2/3 -> Product2/3
  Demux2/2 -> Product4/3
  Demux2/1 -> Product1/3
  c/1 -> Product4/2
  Mux18/1 -> pqr_n/1
  Product1/1 -> Mux18/1
  Saturation/1 -> Product1/1, Product4/1, Product2/1

== system Plant/Actuators/Propulsion Forces and Moments/ESCs ==
  Control_Out : Inport
  Bus Selector : BusSelector  OutputSignals=actuator_cmd
  Constant : Constant  Value=1000  OutDataTypeStr=uint16
  Gain : Gain  Gain=0.001  OutDataTypeStr=single
  Rotor_Delay : Subsystem  mask{K=1, T=T}
      mask Display: disp('K/(1+Tz^{-1})', 'texmode', 'on')
  Rotor_Speed : Subsystem
  Saturation : Saturate  UpperLimit=2000  LowerLimit=1000
  Selector : Selector  InputPortWidth=16  IndexOptions=Index vector (dialog)  Indices=[1:2]  OutputSizes=1
  Subtract : Sum  Inputs=+-  OutDataTypeStr=Inherit: Same as accumulator
  rotor_speed_radPs : Outport
  wires:
  Rotor_Delay/1(out) -> rotor_speed_radPs/1
  Control_Out/1 -> Bus Selector/1
  Gain/1 -> Rotor_Speed/1(u0)
  Rotor_Speed/1(omega_B_radPs) -> Rotor_Delay/1(in)
  Bus Selector/1 -> Selector/1  "<actuator_cmd>"
  Subtract/1 -> Gain/1
  Saturation/1 -> Subtract/1
  Selector/1 -> Saturation/1
  Constant/1 -> Subtract/2

== system Plant/Actuators/Propulsion Forces and Moments/Force ==
  rotor_speed_radPs : Inport
  Constant : Constant  Value=0  OutDataTypeStr=single
  Constant1 : Constant  Value=0  OutDataTypeStr=single
  Mux : Mux  Inputs=3
  Rotor_Thrust : Subsystem  mask{cT=plant_model.Ct}
  Sum of Elements : Sum  Inputs=+
  force_B_N : Outport
  wires:
  rotor_speed_radPs/1 -> Rotor_Thrust/1(rotor_speed_radPs)
  Sum of Elements/1 -> Mux/1
  Rotor_Thrust/1(thrust_B_N) -> Sum of Elements/1
  Mux/1 -> force_B_N/1
  Constant1/1 -> Mux/3
  Constant/1 -> Mux/2

== system Plant/Actuators/Wind_Triangle/Attack_Angle ==
  Va_B : Inport
  Atan : Trigonometry  Operator=atan
  Divide : Product  Inputs=*/
  Saturation : Saturate  UpperLimit=inf  LowerLimit=0.1
  Selector : Selector  InputPortWidth=3  IndexOptions=Index vector (dialog)  Indices=3  OutputSizes=1
  Selector1 : Selector  InputPortWidth=3  IndexOptions=Index vector (dialog)  Indices=1  OutputSizes=1
  alpha_rad : Outport
  wires:
  Va_B/1 -> Selector/1, Selector1/1
  Selector/1 -> Divide/1  "w"
  Selector1/1 -> Saturation/1  "u"
  Divide/1 -> Atan/1
  Atan/1 -> alpha_rad/1
  Saturation/1 -> Divide/2

== system Plant/Actuators/Wind_Triangle/Slide_Angle ==
  Va_B : Inport
  Asin : Trigonometry  Operator=asin
  Divide : Product  Inputs=*/
  Saturation : Saturate  UpperLimit=inf  LowerLimit=0.1
  Selector : Selector  InputPortWidth=3  IndexOptions=Index vector (dialog)  Indices=2  OutputSizes=1
  Vector Modulus : FMT_Model_Lib/Math/Vector Modulus
      settings: SourceProductName=FMT Toolbox
  beta_rad : Outport
  wires:
  Va_B/1 -> Selector/1, Vector Modulus/1
  Selector/1 -> Divide/1
  Vector Modulus/1 -> Saturation/1
  Divide/1 -> Asin/1
  Asin/1 -> beta_rad/1
  Saturation/1 -> Divide/2

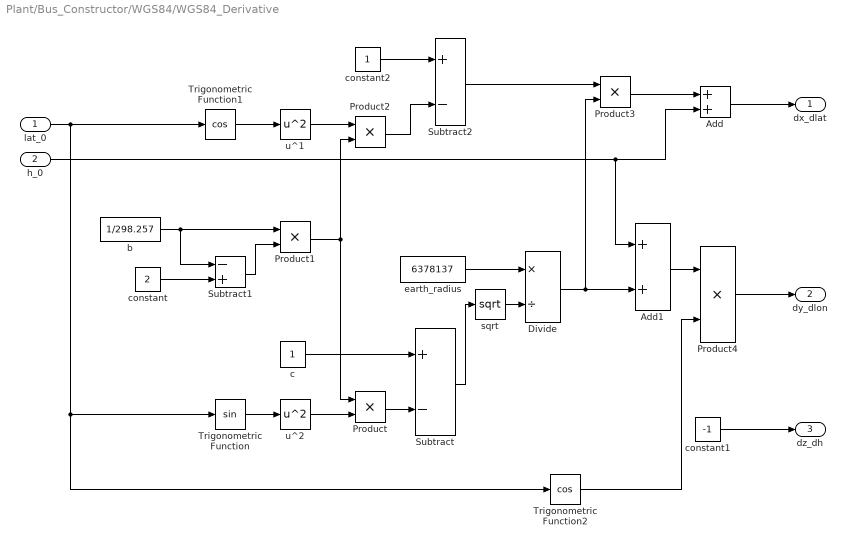
== system Plant/Bus_Constructor/WGS84/WGS84_Derivative ==
  lat_0 : Inport
  h_0 : Inport  Port=2
  Add : Sum
  Add1 : Sum
  Divide : Product  Inputs=*/
  Product{,1..4} (5 alike) : Product  RndMeth=Zero
  Subtract : Sum  Inputs=+-
  Subtract1 : Sum  Inputs=-+
  Subtract2 : Sum  Inputs=+-
  Trigonometric Function : Trigonometry
  Trigonometric Function1 : Trigonometry  Operator=cos
  Trigonometric Function2 : Trigonometry  Operator=cos
  b : Constant  Value=1/298.257
  c : Constant
  constant : Constant  Value=2
  constant1 : Constant  Value=-1
  constant2 : Constant
  earth_radius : Constant  Value=6378137
  sqrt : Math  Operator=sqrt  SaturateOnIntegerOverflow=on
  u^1 : Math  Operator=square  SaturateOnIntegerOverflow=on
  u^2 : Math  Operator=square  SaturateOnIntegerOverflow=on
  dx_dlat : Outport
  dy_dlon : Outport  Port=2
  dz_dh : Outport  Port=3  InitialOutput=1
  wires:
  constant1/1 -> dz_dh/1
  Product4/1 -> dy_dlon/1
  Add1/1 -> Product4/1
  Trigonometric Function2/1 -> Product4/2
  Product3/1 -> Add/1
  Subtract2/1 -> Product3/1
  Product2/1 -> Subtract2/2
  u^1/1 -> Product2/1
  Trigonometric Function1/1 -> u^1/1
  constant2/1 -> Subtract2/1
  h_0/1 -> Add1/1, Add/2
  Add/1 -> dx_dlat/1
  Divide/1 -> Product3/2, Add1/2
  sqrt/1 -> Divide/2
  Product1/1 -> Product2/2, Product/1
  Subtract1/1 -> Product1/2
  constant/1 -> Subtract1/2
  b/1 -> Subtract1/1, Product1/1
  Product/1 -> Subtract/2
  Subtract/1 -> sqrt/1
  c/1 -> Subtract/1
  u^2/1 -> Product/2
  Trigonometric Function/1 -> u^2/1
  lat_0/1 -> Trigonometric Function2/1, Trigonometric Function/1, Trigonometric Function1/1
  earth_radius/1 -> Divide/1

== system Plant/Bus_Constructor/WGS84/Zero_Value_Exclusion ==
  u : Inport
  Abs : Abs
  Constant : Constant
  Product : Product  RndMeth=Zero
  Saturation : Saturate  UpperLimit=10e7  LowerLimit=1e-6  LinearizeAsGain=off
  Sign : Signum
  Switch : Switch  Criteria=u2 ~= 0
  y : Outport
  wires:
  u/1 -> Sign/1, Abs/1
  Abs/1 -> Saturation/1
  Saturation/1 -> Product/1
  Sign/1 -> Switch/2, Switch/1
  Product/1 -> y/1
  Switch/1 -> Product/2
  Constant/1 -> Switch/3

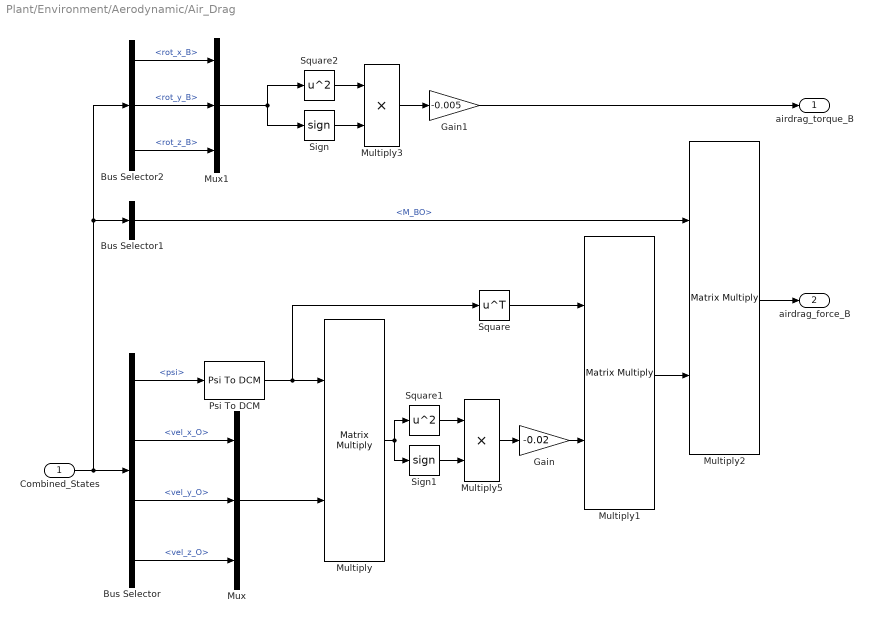
== system Plant/Environment/Aerodynamic/Air_Drag ==
  Combined_States : Inport
  Bus Selector : BusSelector  OutputSignals=Plant_States.psi,Plant_States.vel_x_O,Plant_States.vel_y_O,Plant_States.vel_z_O
  Bus Selector1 : BusSelector  OutputSignals=Extended_States.M_BO
  Bus Selector2 : BusSelector  OutputSignals=Plant_States.rot_x_B,Plant_States.rot_y_B,Plant_States.rot_z_B
  Gain : Gain  Gain=-0.02
  Gain1 : Gain  Gain=-0.005
  Multiply : Product  Multiplication=Matrix(*)
  Multiply1 : Product  Multiplication=Matrix(*)
  Multiply2 : Product  Multiplication=Matrix(*)
  Multiply3 : Product
  Multiply5 : Product
  Mux : Mux  Inputs=3
  Mux1 : Mux  Inputs=3
  Psi To DCM : FMT_Model_Lib/Transformation/Psi To DCM
      settings: SourceProductName=FMT Toolbox
  Sign : Signum
  Sign1 : Signum
  Square : Math  Operator=transpose  SaturateOnIntegerOverflow=on
  Square1 : Math  Operator=square  SaturateOnIntegerOverflow=on
  Square2 : Math  Operator=square  SaturateOnIntegerOverflow=on
  airdrag_torque_B : Outport
  airdrag_force_B : Outport  Port=2
  wires:
  Bus Selector/2 -> Mux/1  "<vel_x_O>"
  Bus Selector/3 -> Mux/2  "<vel_y_O>"
  Gain/1 -> Multiply1/2
  Mux/1 -> Multiply/2
  Combined_States/1 -> Bus Selector2/1, Bus Selector1/1, Bus Selector/1
  Bus Selector/4 -> Mux/3  "<vel_z_O>"
  Multiply/1 -> Sign1/1, Square1/1
  Bus Selector/1 -> Psi To DCM/1  "<psi>"
  Psi To DCM/1 -> Multiply/1, Square/1
  Square/1 -> Multiply1/1
  Multiply1/1 -> Multiply2/2
  Bus Selector1/1 -> Multiply2/1  "<M_BO>"
  Multiply2/1 -> airdrag_force_B/1
  Bus Selector2/1 -> Mux1/1  "<rot_x_B>"
  Bus Selector2/2 -> Mux1/2  "<rot_y_B>"
  Bus Selector2/3 -> Mux1/3  "<rot_z_B>"
  Mux1/1 -> Sign/1, Square2/1
  Gain1/1 -> airdrag_torque_B/1
  Square1/1 -> Multiply5/1
  Square2/1 -> Multiply3/1
  Multiply3/1 -> Gain1/1
  Sign/1 -> Multiply3/2
  Multiply5/1 -> Gain/1
  Sign1/1 -> Multiply5/2

== system Plant/Environment/Collision_Response/Friction_Response ==
  vr_B : Inport
  n_B : Inport  Port=2
  Constant : Constant  Value=0.01  OutDataTypeStr=single
  Divide : Product  Inputs=*/
  Dot Product : DotProduct  InputSameDT=on  OutDataTypeStr=Inherit: Inherit via internal rule
  Dot Product2 : DotProduct  InputSameDT=on  OutDataTypeStr=Inherit: Inherit via internal rule
  Gain3 : Gain  Gain=-plant_model.mass
  Multiply : Product
  Multiply3 : Product
  Multiply4 : Product
  Sum : Sum  Inputs=+-|
  Vector Modulus : FMT_Model_Lib/Math/Vector Modulus
      settings: SourceProductName=FMT Toolbox
  Vector Normalize : FMT_Model_Lib/Math/Vector Normalize
      settings: SourceProductName=FMT Toolbox
  force_B_N : Outport
  wires:
  n_B/1 -> Multiply/2, Vector Modulus/1, Dot Product/2
  Dot Product/1 -> Multiply/1
  Sum/1 -> Vector Normalize/1
  vr_B/1 -> Sum/1, Dot Product2/1, Dot Product/1
  Multiply/1 -> Sum/2
  Multiply3/1 -> Multiply4/2, Dot Product2/2  "t"
  Vector Normalize/1 -> Multiply3/1
  Vector Modulus/1 -> Multiply3/2
  Constant/1 -> Divide/2
  Divide/1 -> Gain3/1
  Gain3/1 -> Multiply4/1
  Dot Product2/1 -> Divide/1
  Multiply4/1 -> force_B_N/1

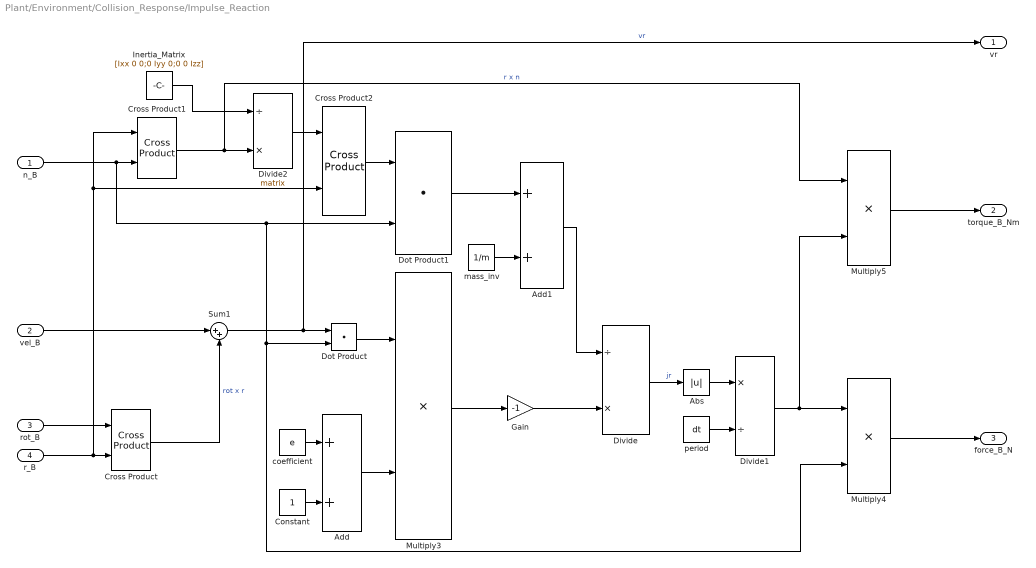
== system Plant/Environment/Collision_Response/Impulse_Reaction ==
  n_B : Inport
  vel_B : Inport  Port=2
  rot_B : Inport  Port=3
  r_B : Inport  Port=4
  Abs : Abs
  Add : Sum
  Add1 : Sum
  Constant : Constant  OutDataTypeStr=single
  Cross Product : FMT_Model_Lib/Math/Cross Product
      settings: SourceProductName=FMT Toolbox
  Cross Product1 : FMT_Model_Lib/Math/Cross Product
      settings: SourceProductName=FMT Toolbox
  Cross Product2 : FMT_Model_Lib/Math/Cross Product
      settings: SourceProductName=FMT Toolbox
  Divide : Product  Inputs=/*
  Divide1 : Product  Inputs=*/
  Divide2 : Product  Inputs=/*  Multiplication=Matrix(*)
  Dot Product : DotProduct  InputSameDT=on  OutDataTypeStr=Inherit: Inherit via internal rule
  Dot Product1 : DotProduct  InputSameDT=on  OutDataTypeStr=Inherit: Inherit via internal rule
  Gain : Gain  Gain=-1
  Inertia_Matrix : Constant  Value=[Ixx 0 0;0 Iyy 0;0 0 Izz]  OutDataTypeStr=single
  Multiply3 : Product
  Multiply4 : Product
  Multiply5 : Product
  Sum1 : Sum  Inputs=|++
  coefficient : Constant  Value=e  OutDataTypeStr=single
  mass_inv : Constant  Value=1/m  OutDataTypeStr=single
  period : Constant  Value=dt  OutDataTypeStr=single
  vr : Outport
  torque_B_Nm : Outport  Port=2
  force_B_N : Outport  Port=3
  wires:
  Divide/1 -> Abs/1  "jr"
  mass_inv/1 -> Add1/2
  Cross Product2/1 -> Dot Product1/1
  coefficient/1 -> Add/1
  r_B/1 -> Cross Product1/1, Cross Product2/2, Cross Product/2
  Add/1 -> Multiply3/2
  n_B/1 -> Dot Product/2, Multiply4/2, Dot Product1/2, Cross Product1/2
  Cross Product/1 -> Sum1/2  "rot x r"
  Sum1/1 -> vr/1, Dot Product/1  "vr"
  Gain/1 -> Divide/2
  Constant/1 -> Add/2
  period/1 -> Divide1/2
  Add1/1 -> Divide/1
  Divide1/1 -> Multiply4/1, Multiply5/2
  Multiply3/1 -> Gain/1
  Divide2/1 -> Cross Product2/1
  Inertia_Matrix/1 -> Divide2/1
  Cross Product1/1 -> Multiply5/1, Divide2/2  "r x n"
  Dot Product1/1 -> Add1/1
  Dot Product/1 -> Multiply3/1
  rot_B/1 -> Cross Product/1
  vel_B/1 -> Sum1/1
  Multiply5/1 -> torque_B_Nm/1
  Multiply4/1 -> force_B_N/1
  Abs/1 -> Divide1/1

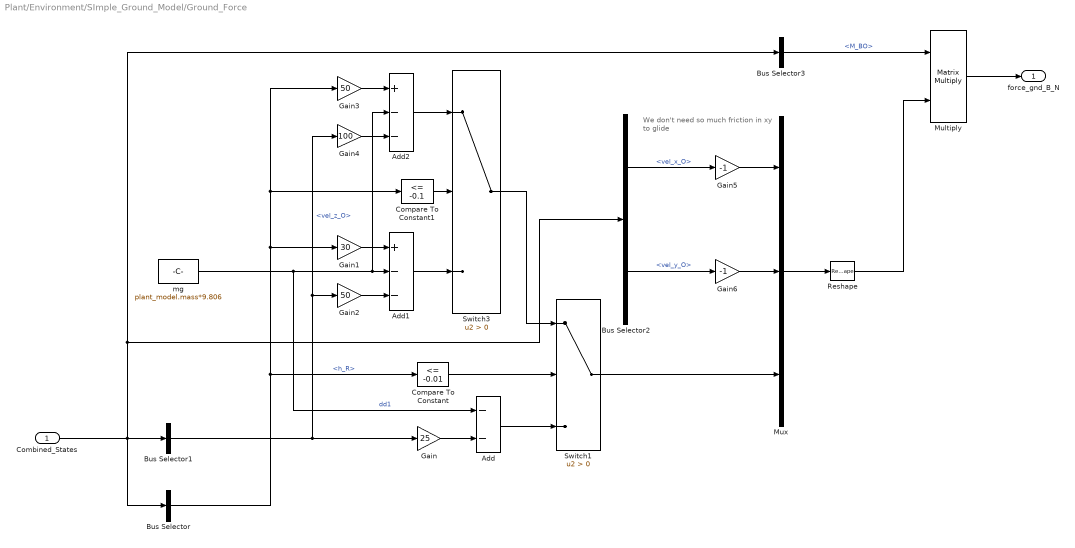
== system Plant/Environment/SImple_Ground_Model/Ground_Force ==
  note: We don't need so much
      | friction in xy to glide
  Combined_States : Inport
  Add : Sum  Inputs=--
  Add1 : Sum  Inputs=+--
  Add2 : Sum  Inputs=+--
  Bus Selector : BusSelector  OutputSignals=Plant_States.h_R
  Bus Selector1 : BusSelector  OutputSignals=Plant_States.vel_z_O
  Bus Selector2 : BusSelector  OutputSignals=Plant_States.vel_x_O,Plant_States.vel_y_O
  Bus Selector3 : BusSelector  OutputSignals=Extended_States.M_BO
  Compare To Constant : simulink/Logic and Bit Operations/Compare To Constant  relop=<=  const=-0.01  OutDataTypeStr=boolean
  Compare To Constant1 : simulink/Logic and Bit Operations/Compare To Constant  relop=<=  const=-0.1  OutDataTypeStr=boolean
  Gain : Gain  Gain=25
  Gain1 : Gain  Gain=30
  Gain2 : Gain  Gain=50
  Gain3 : Gain  Gain=50
  Gain4 : Gain  Gain=100
  Gain5 : Gain  Gain=-1
  Gain6 : Gain  Gain=-1
  Multiply : Product  Multiplication=Matrix(*)
  Mux : Mux  Inputs=3
  Reshape : Reshape  OutputDimensionality=Customize  OutputDimensions=[3,1]
  Switch1 : Switch  Criteria=u2 > Threshold
  Switch3 : Switch  Criteria=u2 > Threshold
  mg : Constant  Value=plant_model.mass*9.806  OutDataTypeStr=single
  force_gnd_B_N : Outport
  wires:
  Switch1/1 -> Mux/3
  Bus Selector/1 -> Compare To Constant/1, Gain1/1, Gain3/1, Compare To Constant1/1  "<h_R>"
  Bus Selector1/1 -> Gain4/1, Gain2/1, Gain/1  "<vel_z_O>"
  Switch3/1 -> Switch1/1
  Gain1/1 -> Add1/1
  Gain5/1 -> Mux/1
  Gain3/1 -> Add2/1
  Compare To Constant/1 -> Switch1/2
  mg/1 -> Add/1, Add2/2, Add1/2  "dd1"
  Gain/1 -> Add/2
  Bus Selector2/2 -> Gain6/1  "<vel_y_O>"
  Gain2/1 -> Add1/3
  Add/1 -> Switch1/3
  Add2/1 -> Switch3/1
  Bus Selector2/1 -> Gain5/1  "<vel_x_O>"
  Gain6/1 -> Mux/2
  Compare To Constant1/1 -> Switch3/2
  Gain4/1 -> Add2/3
  Add1/1 -> Switch3/3
  Bus Selector3/1 -> Multiply/1  "<M_BO>"
  Mux/1 -> Reshape/1
  Multiply/1 -> force_gnd_B_N/1
  Reshape/1 -> Multiply/2
  Combined_States/1 -> Bus Selector/1, Bus Selector1/1, Bus Selector3/1, Bus Selector2/1
